simulink model "lr5_v20_part2"  (R2023a)
settings: Solver=ode45  StartTime=0.0  StopTime=2  MaxStep=0.001  RelTol=1e-8  AbsTol=1e-10
undefined symbols (not defined in the file): K1
settings Model: Creator=theju  LastModifiedBy=theju

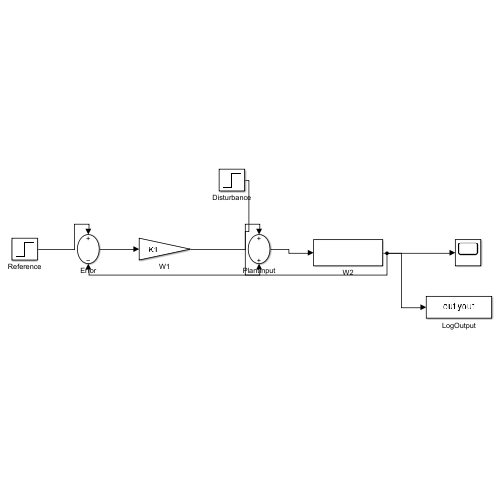
[thumbnail: Simulink's stored preview of the top-level diagram]
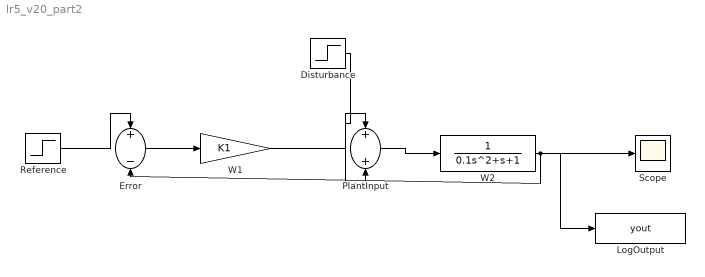
== system lr5_v20_part2 ==
  Disturbance : Step  Time=0  After=0  SampleTime=0
  Error : Sum  Inputs=+-
  LogOutput : ToWorkspace  VariableName=yout  SaveFormat=Timeseries  SampleTime=-1
  PlantInput : Sum
  Reference : Step  Time=0  SampleTime=0
  Scope : Scope
  W1 : Gain  Gain=K1
  W2 : TransferFcn  Denominator=[0.1 1 1]
  wires:
  Reference/1 -> Error/1
  W2/1 -> Error/2, Scope/1, LogOutput/1
  Error/1 -> W1/1
  W1/1 -> PlantInput/1
  Disturbance/1 -> PlantInput/2
  PlantInput/1 -> W2/1
